simulink model "Dynamics_UCS"  (R2026a)
settings: Solver=FixedStepDiscrete  StopTime=S.tspan  FixedStep=S.dt_sim  RelTol=rel_tol  AbsTol=abs_tol
StopFcn:
  | defaultToFileBlockNames(bdroot);
undefined symbols (not defined in the file): I, S
PreSaveFcn:
  | defaultToFileBlockNames(bdroot);
settings Model: Creator=koryh  LastModifiedBy=kjhaydon

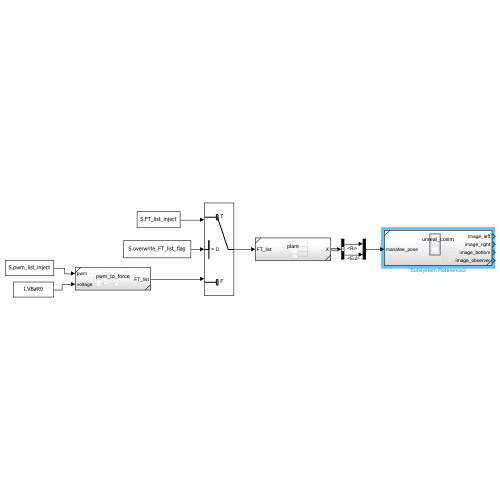
[thumbnail: Simulink's stored preview of the top-level diagram]
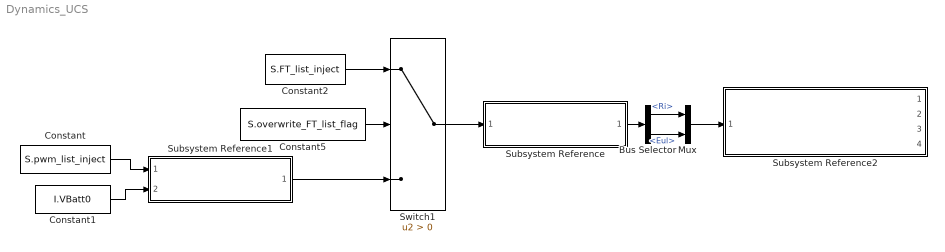
== system Dynamics_UCS ==
  Bus Selector : BusSelector  OutputSignals=Ri,Eul
  Constant : Constant  Value=S.pwm_list_inject
  Constant1 : Constant  Value=I.VBatt0
  Constant2 : Constant  Value=S.FT_list_inject
  Constant5 : Constant  Value=S.overwrite_FT_list_flag
  Mux : Mux  Inputs=2
  Subsystem Reference : Subsystem  ReferencedSubsystem=plant
  Subsystem Reference1 : Subsystem  ReferencedSubsystem=pwm_to_force
  Subsystem Reference2 : Subsystem  ReferencedSubsystem=unreal_cosim
  Switch1 : Switch  Criteria=u2 > Threshold  SaturateOnIntegerOverflow=off  InputSameDT=off
  wires:
  Subsystem Reference/1 -> Bus Selector/1
  Bus Selector/1 -> Mux/1  "<Ri>"
  Bus Selector/2 -> Mux/2  "<Eul>"
  Switch1/1 -> Subsystem Reference/1
  Constant/1 -> Subsystem Reference1/1
  Constant1/1 -> Subsystem Reference1/2
  Mux/1 -> Subsystem Reference2/1
  Constant2/1 -> Switch1/1
  Subsystem Reference1/1 -> Switch1/3
  Constant5/1 -> Switch1/2
